simulink model "sf_pool"  (R2025b)
settings: Solver=ode45  StartTime=0.0  StopTime=10  MaxStep=.1  RelTol=1e-3  EnableMultiTasking=on
model workspace (MATLAB code in the model file):
  | kp = 100000;
  | kv = 40;
  | kfriction = 10;
  | tableLen = 44;
  | tableWidth = 22;
  | ballRadius = 1;
  | N = 16;
CloseFcn:
  | sf_pool_plotter('close');
settings Model: ExtModeAutoUpdateStatusClock=off  Creator=The MathWorks, Inc.  LastModifiedBy=The MathWorks, Inc.
settings SolverCC: ConsecutiveZCsStepRelTol=1e-3  AlgebraicLoopSolver=TrustRegion  InsertRTBMode=Auto
settings DataIOCC: LimitDataPoints=on  SaveFormat=Array  ReturnWorkspaceOutputs=off
settings OptimizationCC: ReuseModelBlockBuffer=off  ExpressionDepthLimit=2147483647.0  InitFltsAndDblsToZero=on  LifeSpan=inf
settings DebuggingCC: UnderspecifiedInitializationDetection=Classic  MergeDetectMultiDrivingBlocksExec=none  SolverPrmCheckMsg=warning  FcnCallInpInsideContextMsg=warning  UnconnectedInputMsg=warning  UnconnectedOutputMsg=warning  UnconnectedLineMsg=warning  AllowSymbolicDim=off  StateNameClashWarn=warning  SFUnexpectedBacktrackingDiag=warning  SFNoUnconditionalDefaultTransitionDiag=warning  SFExecutionAtInitializationDiag=none  ArithmeticOperatorsInVariantConditions=warning
settings HardwareCC: ProdBitPerPointer=32.0  ProdBitPerSizeT=32.0  ProdBitPerPtrDiffT=32.0  ProdLargestAtomicFloat=None  ProdIntDivRoundTo=Undefined  ProdEndianess=Unspecified  ProdWordSize=32.0  ProdHWDeviceType=32-bit Generic
settings ModelReferenceCC: EnableRefExpFcnMdlSchedulingChecks=on  PropagateSignalLabelsOutOfModel=off
settings SFSimCC: SFSimEcho=off  SimUseLocalCustomCode=off  SimParseCustomCode=off  CustomCodeUndefinedFunction=UseInterfaceOnly
settings RTWCC: RTWUseLocalCustomCode=off  GPUComputeCapability=3.5
settings CodeAppCC: StateflowObjectComments=on
settings GRTTargetCC: TargetLangStandard=C89/C90 (ANSI)  CombineOutputUpdateFcns=off  GRTInterface=on
settings ConfigComp: CovMetricSettings=dw  CovSaveCumulativeToWorkspaceVar=on  CovSaveSingleToWorkspaceVar=on  CovExternalEMLEnable=off  CovSFcnEnable=off

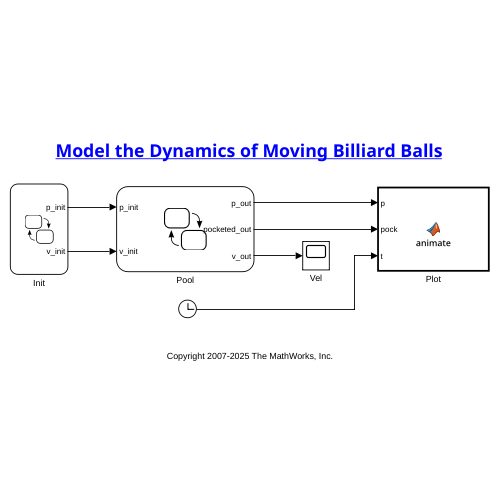
[thumbnail: Simulink's stored preview of the top-level diagram]
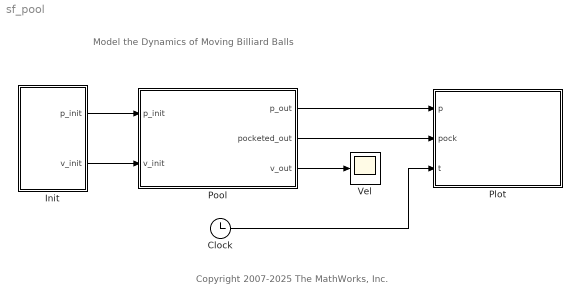
== system sf_pool ==
  note: Copyright 2007-2025 The MathWorks, Inc.
  note: Model the Dynamics of Moving Billiard Balls
  Clock : Clock
  Init : Stateflow chart  TreatAsAtomicUnit=on
  Plot : MATLAB Function  TreatAsAtomicUnit=on
  Pool : Stateflow chart  TreatAsAtomicUnit=on
  Vel : Scope
  wires:
  Pool/1(p_out) -> Plot/1(p)
  Pool/2(pocketed_out) -> Plot/2(pock)
  Init/1(p_init) -> Pool/1(p_init)
  Init/2(v_init) -> Pool/2(v_init)
  Clock/1 -> Plot/3(t)
  Pool/3(v_out) -> Vel/1

== stateflow chart sf_pool/Init ==
  state A
  (default) -> A : {init();}
  data: p_init output double size=[N 2]; v_init output double size=[N 2]; N parameter
  function init:
    | function init
    | coder.extrinsic('sf_pool_plotter_3d', 'sf_pool_plotter');
    | 
    | [p_init, v_init] = sf_pool_plotter('init', zeros(N,2), zeros(N,2));

== stateflow chart sf_pool/Pool ==
  settings: updateMethod=CONTINUOUS
  state TotalDynamics
    du:
    % derivatives
    p_dot = v;
    v_dot = frictionForce() + interactionForce();
    % chart outputs
    p_out = p;
    v_out = v;
    pocketed_out = pocketed;
  TotalDynamics -> TotalDynamics [order 1] : [isAnyBallGoingToStop()]
      | {updateStopFlags();}
  TotalDynamics -> TotalDynamics [order 2] : [hasBallInteractionChanged()]
      | {ball_interaction = getBallInteraction();
      |  updateStopFlags();}
  (default) -> TotalDynamics : {initBalls();}
  TotalDynamics -> TotalDynamics [order 3] : [isAnyBallNewlyPocketed()]
      | {pocketNewBalls();
      |  updateStopFlags();}
  TotalDynamics -> TotalDynamics [order 4] : [isAnyBallOutOfBounds()]
      | {resetBallsPosAndVel();
      |  updateStopFlags();}
  data: f function_output double size=size(p); f function_output double size=[N 2]; yn function_output double; yn function_output double; yn function_output double; yn function_output boolean; pp function_input double size=[1 2]; yn function_output boolean; balli function_output boolean size=[N N]; ball_interaction local boolean size=[N N]; p local double size=[N 2]; v local double size=[N 2]; kp parameter double; ballRadius parameter double; pocketed local boolean size=N; p_out output double size=size(p); pocketed_out output boolean size=size(pocketed); v_out output double size=size(v); tableLen parameter double; tableWidth parameter double; kv parameter double; last_vel local double size=size(v); stopped local boolean size=N; kfriction parameter double; p_init input double size=size(p); v_init input double size=size(p); N parameter
  data p settings: updateMethod=SF_CONTINUOUS_TIME_DATA
  data v settings: updateMethod=SF_CONTINUOUS_TIME_DATA
  function initBalls:
    | function initBalls
    | 
    | p = p_init;
    | v = v_init;
    | 
    | % x_off = 20;
    | % y_off = 0;
    | % n = 1;
    | % for i=1:5
    | %     for j=1:i
    | %         p(n,1) = x_off;
    | %         p(n,2) = y_off + (j-1)*2*ballRadius;
    | %         n = n + 1;
    | %     end
    | %     x_off = x_off + 2*ballRadius*cos(pi/6);
    | %     y_off = y_off - 2*ballRadius*sin(pi/6);
    | % end
    | % 
    | % p(n,1) = initXPos;
    | % p(n,2) = initYPos;
    | % 
    | % v = zeros(N,2);
    | % v(n,1) = initXVel;
    | % v(n,2) = initYVel;
    | 
    | stopped = true(N,1);
    | stopped(end) = false;
    | 
    | pocketed = false(N,1);
    | ball_interaction = false(N, N);
    | 
    | last_vel = v;
  function f = frictionForce:
    | function f = frictionForce
    | % This function calculates the forces on the balls due to friction from the
    | % table. We use a simple constant friction force model between the ball
    | % and the table.
    | 
    | f = zeros(N,2);
    | for i=1:N
    |     if stopped(i)
    |        continue
    |     else
    |         % Note that we are using last_vel to calculate the direction of 
    |         % the friction force because we are guaranteed that 
    |         % |last_vel(i,:)| is large when stopped(i) is false. We cannot
    |         % use v(i,:) directly because this function gets called in minor
    |         % time steps and v(i,:) can become very small at some minor time 
    |         % step even if it was large at the previous major time-step. 
    |         f(i,:) = -kfriction*last_vel(i,:)/norm(last_vel(i,:)); %#ok
    |     end
    | end
  function f = interactionForce:
    | function f = interactionForce
    | % given the positions and velocities of all the balls, we want to find out 
    | % the interaction force between the various balls
    | 
    | f = zeros(N,2);
    | for i=1:(N-1)
    |     if pocketed(i)
    |         continue;
    |     end
    |     for j=(i+1):N
    |         if pocketed(j)
    |             continue;
    |         end
    |         if ball_interaction(i,j)
    |             dp = p(i,:)-p(j,:);
    |             dv = v(i,:)-v(j,:);
    |             fr = kp*(2*ballRadius-norm(dp))*dp/norm(dp) + ...
    |                  -kv*dv;
    |             f(i,:) = f(i,:) + fr;
    |             f(j,:) = f(j,:) - fr;
    |         end
    |     end
    | end
  function yn = isAnyBallGoingToStop:
    | function yn = isAnyBallGoingToStop
    | 
    | for i=1:N
    |     if v(i,:)*last_vel(i,:)' < 0
    |         yn = 1;
    |         return
    |     end
    | end
    | yn = 0;
  function yn = hasBallInteractionChanged:
    | function yn = hasBallInteractionChanged
    | if ~isequal(ball_interaction, getBallInteraction())
    |     yn = 1;
    | else
    |     yn = 0;
    | end
  function yn = isAnyBallNewlyPocketed:
    | function yn = isAnyBallNewlyPocketed
    |  
    | for i=1:N
    |     if pocketed(i)
    |         continue;
    |     end
    |     if nearHole(p(i,:))
    |         yn = 1;
    |         return
    |     end
    | end
    | yn = 0;
  function yn = isAnyBallOutOfBounds:
    | function yn = isAnyBallOutOfBounds
    | for i=1:N
    |     if p(i,1) < -tableLen || p(i,1) > tableLen || ...
    |        p(i,2) < -tableWidth || p(i,2) > tableWidth
    |         yn = true;
    |         return;
    |     end
    | end
    | yn = false;
  function yn = nearHole(pp):
    | function yn = nearHole(pp)
    | % first reflect the ball into the upper right quadrant. The check becomes
    | % slightly faster then.
    | pp = abs(pp);
    | if norm(pp-[tableLen, tableWidth]) < 1.2*ballRadius
    |     yn = true;
    | elseif norm(pp-[0, tableWidth]) < ballRadius
    |     yn = true;
    | else
    |     yn = false;
    | end
  function balli = getBallInteraction:
    | function balli = getBallInteraction
    | 
    | balli = false(N,N);
    | for i=1:(N-1)
    |     for j=(i+1):N
    |         if norm(p(i,:)-p(j,:)) < 2*ballRadius
    |             balli(i,j) = true;
    |         else
    |             balli(i,j) = false;
    |         end
    |     end
    | end
  function updateStopFlags:
    | function updateStopFlags
    | 
    | for i=1:N
    |     if norm(v(i,:)) < 1e-3
    |         stopped(i) = true;
    |     elseif norm(v(i,:)) > 1e-3
    |         stopped(i) = false;
    |     end
    | end
    | last_vel = v;
  function pocketNewBalls:
    | function pocketNewBalls
    | for i=1:N
    |     if pocketed(i)
    |         continue;
    |     end
    |     if nearHole(p(i,:))
    |         pocketed(i) = true;
    |         v(i,:) = zeros(1,2);
    |     end
    | end
  function resetBallsPosAndVel:
    | function resetBallsPosAndVel
    | 
    | for i=1:N
    |     if p(i,1) < -tableLen
    |         p(i,1) = -2*tableLen-p(i,1);
    |         v(i,1) = -0.8*v(i,1);
    |         v(i,2) = 0.8*v(i,2);
    |     elseif p(i,1) > tableLen
    |         p(i,1) = 2*tableLen-p(i,1);
    |         v(i,1) = -0.8*v(i,1);
    |         v(i,2) = 0.8*v(i,2);
    |     end
    |     if p(i,2) < -tableWidth
    |         p(i,2) = -2*tableWidth-p(i,2);
    |         v(i,2) = -0.8*v(i,2);
    |         v(i,1) = 0.8*v(i,1);
    |     elseif p(i,2) > tableWidth
    |         p(i,2) = 2*tableWidth-p(i,2);
    |         v(i,2) = -0.8*v(i,2);
    |         v(i,1) = 0.8*v(i,1);
    |     end
    | end

== matlab function sf_pool/Plot ==
  settings: updateMethod=DISCRETE  sampleTime=.03
  data: p input; pock input; t input
function animate(p, pock, t)
%#codegen

coder.extrinsic('sf_pool_plotter', 'sf_pool_plotter_3d');

sf_pool_plotter('draw', p, pock, t);
